simulink model "liquid_cooling_phase_a"  (R2026a)
settings: Solver=ode23t  StopTime=p.stopTime  MaxStep=1  RelTol=1e-5
model workspace (MAT data in the model file):
  p.Tambient_C = 25
  p.Tset_C = 40
  p.Tinitial_K = 298.15
  p.mChip = 0.16
  p.cpChip = 500
  p.mWater = 0.1
  p.cpWater = 4180
  p.RchipWater = 0.1
  p.Gpassive = 0.4
  p.Gfan = 5
  p.tauFan = 2
  p.Kp = 0.24
  p.Ki = 0.0012
  p.Kd = 0.5
  p.N = 1
  p.Qinitial = 20
  p.Qfinal = 40
  p.stepTime = 600
  p.stopTime = 1800
values from neighbouring files (symbols this model uses):
  p = getVariable(ws,'p'); p.Kp=g(1); p.Ki=g(2); p.Kd=g(3)    [apply_phase_a_pid_tuning.m]    (also in build_phase_a.m = phase_a_parameters(); phase_a_results.mat = ; pid_tuning_trials.mat = ; run_phase_a.m = getVariable(ws,'p'))
libraries: fl_lib x9, nesl_utility x5, slpidlib x1
settings Model: Creator=Aaron Xu  LastModifiedBy=Aaron Xu

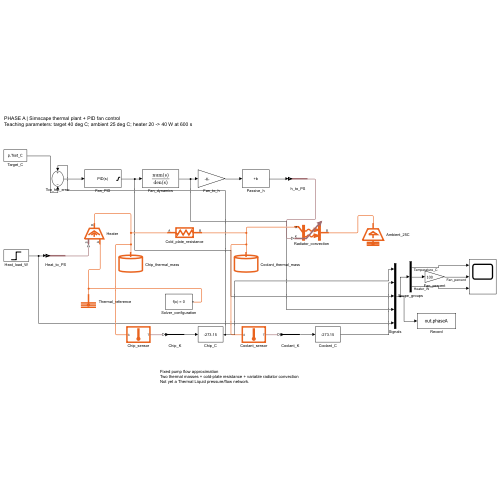
[thumbnail: Simulink's stored preview of the top-level diagram]
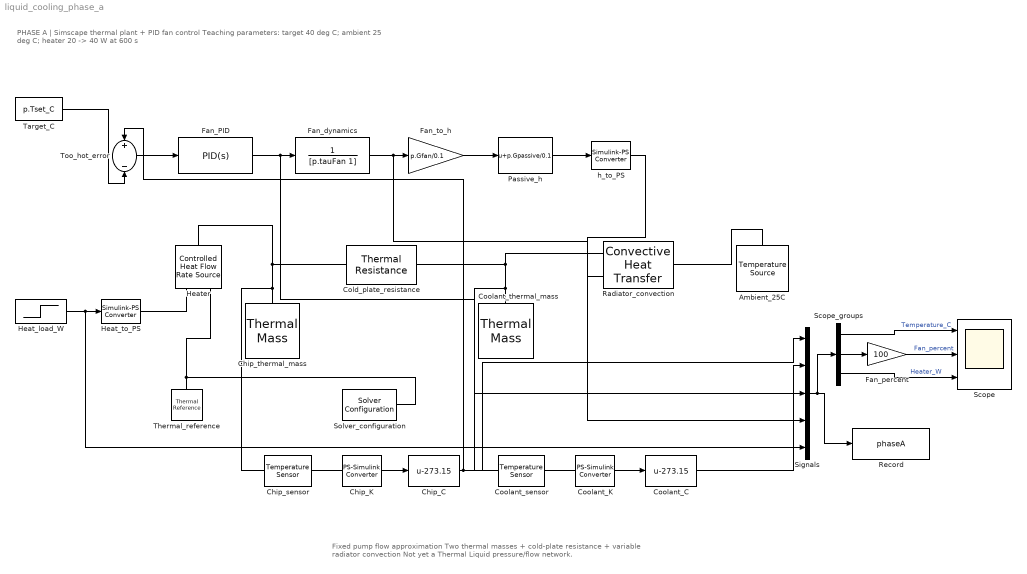
== system liquid_cooling_phase_a ==
  note: PHASE A | Simscape thermal plant + PID fan control
      | Teaching parameters: target 40 deg C; ambient 25 deg C; heater 20 -> 40 W at 600 s
  note: Fixed pump flow approximation
      | Two thermal masses + cold-plate resistance + variable radiator convection
      | Not yet a Thermal Liquid pressure/flow network.
  Ambient_25C : fl_lib/Thermal/Thermal Sources/Temperature Source  temperature=p.Tambient_C+273.15 K
  Chip_C : Bias  Bias=-273.15  SaturateOnIntegerOverflow=off
  Chip_K : nesl_utility/PS-Simulink Converter  PhysicalDomain=network_engine_domain  SubClassName=ps_output  LeftPortType=input  RightPortType=output  PseudoPeriodic=off  Frequencies=[]  VectorFormat=inherit  Unit=K  AffineConversion=off
  Chip_sensor : fl_lib/Thermal/Thermal Sensors/Temperature Sensor  temperature_measure=2
  Chip_thermal_mass : fl_lib/Thermal/Thermal Elements/Thermal Mass  mass_type=foundation.enum.constant_variable.constant  mass=p.mChip kg  sp_heat=p.cpChip J/(K*kg)  mass_min=1e-6 kg  num_ports=foundation.enum.numPorts2.one  m_specify=off  m_priority=High  m=1 kg  m_nominal_specify=off  m_nominal_value=1  m_nominal_unit=kg  T_specify=on  T_priority=High  T=p.Tinitial_K K  T_nominal_specify=off  T_nominal_value=1  T_nominal_unit=K  Q_specify=off  Q_priority=None  Q=0 W  Q_nominal_specify=off  Q_nominal_value=1  Q_nominal_unit=W
  Cold_plate_resistance : fl_lib/Thermal/Thermal Elements/Thermal Resistance  resistance=p.RchipWater K/W  T_specify=off  T_priority=None  T=0 K  T_nominal_specify=off  T_nominal_value=1  T_nominal_unit=K  Q_specify=off  Q_priority=None  Q=0 W  Q_nominal_specify=off  Q_nominal_value=1  Q_nominal_unit=W
  Coolant_C : Bias  Bias=-273.15  SaturateOnIntegerOverflow=off
  Coolant_K : nesl_utility/PS-Simulink Converter  PhysicalDomain=network_engine_domain  SubClassName=ps_output  LeftPortType=input  RightPortType=output  PseudoPeriodic=off  Frequencies=[]  VectorFormat=inherit  Unit=K  AffineConversion=off
  Coolant_sensor : fl_lib/Thermal/Thermal Sensors/Temperature Sensor  temperature_measure=2
  Coolant_thermal_mass : fl_lib/Thermal/Thermal Elements/Thermal Mass  mass_type=foundation.enum.constant_variable.constant  mass=p.mWater kg  sp_heat=p.cpWater J/(K*kg)  mass_min=1e-6 kg  num_ports=foundation.enum.numPorts2.one  m_specify=off  m_priority=High  m=1 kg  m_nominal_specify=off  m_nominal_value=1  m_nominal_unit=kg  T_specify=on  T_priority=High  T=p.Tinitial_K K  T_nominal_specify=off  T_nominal_value=1  T_nominal_unit=K  Q_specify=off  Q_priority=None  Q=0 W  Q_nominal_specify=off  Q_nominal_value=1  Q_nominal_unit=W
  Fan_PID : slpidlib/PID Controller  Controller=PID  Form=Parallel  TimeDomain=Continuous-time  UseExternalTs=off  SampleTime=-1  IntegratorMethod=Forward Euler  FilterMethod=Forward Euler  ControllerParametersSource=internal  P=p.Kp  I=p.Ki  UseKiTs=off  D=p.Kd  UseExternalDerivativeSource=off  N=p.N  UseFilter=on  TunerSelectOption=Transfer Function Based (PID Tuner App)  InitialConditionSource=internal  InitialConditionForIntegrator=0  InitialConditionForFilter=0  DifferentiatorICPrevScaledInput=0  ExternalReset=none  TrackingMode=off  Kt=1  LimitOutput=on  SatLimitsSource=internal  UpperSaturationLimit=1  LowerSaturationLimit=0  LinearizeAsGain=on  AntiWindupMode=clamping  Kb=1  LimitIntegrator=off  UpperIntegratorSaturationLimit=inf  LowerIntegratorSaturationLimit=-inf  POutMin=[]  POutMax=[]  IOutMin=[]  IOutMax=[]  DOutMin=[]  DOutMax=[]  NOutMin=[]  NOutMax=[]  SumOutMin=[]  SumOutMax=[]  SaturationOutMin=[]  SaturationOutMax=[]  PParamMin=[]  PParamMax=[]  IParamMin=[]  IParamMax=[]  DParamMin=[]  DParamMax=[]  NParamMin=[]  NParamMax=[]  KbParamMin=[]  KbParamMax=[]  KtParamMin=[]  KtParamMax=[]  KbOutMin=[]  KbOutMax=[]  KtOutMin=[]  KtOutMax=[]  IntegratorOutMin=[]  IntegratorOutMax=[]  FilterOutMin=[]  FilterOutMax=[]  SumI1OutMin=[]  SumI1OutMax=[]  SumI2OutMin=[]  SumI2OutMax=[]  SumI3OutMin=[]  SumI3OutMax=[]  SumI4OutMin=[]  SumI4OutMax=[]  SumDOutMin=[]  SumDOutMax=[]  DifferentiatorOutMin=[]  DifferentiatorOutMax=[]  FilterDiffOutCoefMin=[]  FilterDiffOutCoefMax=[]  ReciprocalOutMin=[]  ReciprocalOutMax=[]  SumDenOutMin=[]  SumDenOutMax=[]  SumNumOutMin=[]  SumNumOutMax=[]  DivideOutMin=[]  DivideOutMax=[]  UdiffTsProdOutMin=[]  UdiffTsProdOutMax=[]  NTsProdOutMin=[]  NTsProdOutMax=[]  UintegralTsProdOutMin=[]  UintegralTsProdOutMax=[]  UngainTsProdOutMin=[]  UngainTsProdOutMax=[]  ClampingZeroOutDataTypeStr=Inherit: Inherit via back propagation  ClampingZeroOutMin=[]  ClampingZeroOutMax=[]  FilterDenConstantOutDataTypeStr=Inherit: Inherit via back propagation  FilterDenConstantOutMin=[]  FilterDenConstantOutMax=[]  PCopyOutDataTypeStr=Inherit: Inherit via back propagation  PCopyOutMin=[]  PCopyOutMax=[]  NCopyOutDataTypeStr=Inherit: Inherit via back propagation  NCopyOutMin=[]  NCopyOutMax=[]  IntegratorContinuousStateAttributes=''  IntegratorStateMustResolveToSignalObject=off  IntegratorRTWStateStorageClass=Auto  FilterContinuousStateAttributes=''  FilterStateMustResolveToSignalObject=off  FilterRTWStateStorageClass=Auto  ParallelPVariant=InternalParameters  IdealPVariant=Disabled  IVariant=InternalParameters  DVariant=InternalParameters  IntegratorVariant=Continuous  SatVariant=Enabled  AWVariant=ContClampingParallel  PCopyVariant=Disabled  TRVariant=Disabled  FdbkBlocksVariant=Forward  IdealPFdbkVariant=Disabled  SatFdbkVariant=Disabled  DerivativeFilterVariant=ContFilter  NVariant=InternalParameters  NCopyVariant=Disabled  FilterICVariant=InternalICsFilter  IntegratorICVariant=InternalICs  ExternalResetVariant=Disabled  TRSumVariant=Passthrough  SumFdbkVariant=Disabled  SumVariant=Sum_PID  TsampFilterVariant=InternalTs  TsampNgainVariant=Passthrough  TsampIntegralVariant=Disabled_SignalSpec  ExternalSaturationOutDataTypeStr=Inherit: Same as second input  DerivativeSourceVariant=ErrorSignal  PreIntVariant=InternalPreInt
  Fan_dynamics : TransferFcn  Numerator=1  Denominator=[p.tauFan 1]
  Fan_percent : Gain  Gain=100
  Fan_to_h : Gain  Gain=p.Gfan/0.1
  Heat_load_W : Step  Time=p.stepTime  InitialValue=p.Qinitial  FinalValue=p.Qfinal  SampleTime=0
  Heat_to_PS : nesl_utility/Simulink-PS Converter  PhysicalDomain=network_engine_domain  SubClassName=ps_input  LeftPortType=input  RightPortType=output  PseudoPeriodic=off  Frequencies=[]  NoiseDistribution=none  NoiseParameters=[]  Unit=W  AffineConversion=off  FilteringAndDerivatives=provide  SimscapeFilterOrder=1  InputFilterTimeConstant=0.001  UdotUserProvided=0
  Heater : fl_lib/Thermal/Thermal Sources/Controlled Heat Flow Rate Source
  Passive_h : Bias  Bias=p.Gpassive/0.1  SaturateOnIntegerOverflow=off
  Radiator_convection : fl_lib/Thermal/Thermal Elements/Convective Heat Transfer  thermal_type=2  area=0.1 m^2  heat_tr_coeff=20 W/(K*m^2)  min_heat_tr_coeff=1e-3 W/(K*m^2)  T_specify=off  T_priority=None  T=0 K  T_nominal_specify=off  T_nominal_value=1  T_nominal_unit=K  Q_specify=off  Q_priority=None  Q=0 W  Q_nominal_specify=off  Q_nominal_value=1  Q_nominal_unit=W
  Record : ToWorkspace  VariableName=phaseA  SaveFormat=Timeseries  SampleTime=-1
  Scope : Scope  NumInputPorts=3
      settings: TimeSpan=1800  Title=Temperature: channel 1 = chip, channel 2 = coolant  ActiveDisplayYMinimum=24  ActiveDisplayYMaximum=46  YLabel=deg C
  Scope_groups : Demux  Outputs=[2 2 1]
  Signals : Mux  Inputs=5
  Solver_configuration : nesl_utility/Solver Configuration  PhysicalDomain=network_engine_domain  SubClassName=solver  LeftPortType=input  RightPortType=generic  Tones=[]  Harmonics=[]  SimulateNoise=off  Profile=off  UseLocalSampling=off  EnableSwitchedLinearOptims=on  FrequencyDomain=off  UseCCode=off  RelTol=0.001  AbsTol=0.001  MinStep=1e-09  ToWorkspace=off  RevertToSquareIcSolve=off  NumHomotopyIterations=100  PhasorMode=off  PhasorModeNumHarmonics=1  ConsistencySolver=NEWTON_XTOL_AFTER_FTOL  CanonicalOrdering=CANONICAL  OptimizeIntermediates=OPTIMIZED  IndexReductionMethod=DerivativeReplacement  DoDC=off  ResidualTolerance=1e-09  ConsistencyTolSource=GLOBAL  ConsistencyAbsTol=0.001  ConsistencyRelTol=0.001  ConsistencyTolFactor=0.001  UseLocalSolver=off  LocalSolverChoice=NE_BACKWARD_EULER_ADVANCER  ResolveIndetEquations=on  FunctionEvalNumThread=1  LocalSolverSampleTime=0.001  DoFixedCost=off  MaxNonlinIter=3  MaxModeIter=2  ComputeImpulses=off  ImpulseIterations=2  LinearAlgebra=auto  LinearAlgebraNumThread=0  EquationFormulation=NE_TIME_EF  DelaysMemoryBudget=1024  AutomaticFiltering=on  FilteringTimeConstant=0.001  PartitionStorageMethod=AS_NEEDED  PartitionMemoryBudget=1024  PartitionMethod=ROBUST  MultibodyUseLocalSolver=off  MultibodyLocalSolverChoice=ODE1  MultibodyLocalSolverSampleTime=0.001
  Target_C : Constant  Value=p.Tset_C
  Thermal_reference : fl_lib/Thermal/Thermal Elements/Thermal Reference
  Too_hot_error : Sum  Inputs=+-
  h_to_PS : nesl_utility/Simulink-PS Converter  PhysicalDomain=network_engine_domain  SubClassName=ps_input  LeftPortType=input  RightPortType=output  PseudoPeriodic=off  Frequencies=[]  NoiseDistribution=none  NoiseParameters=[]  Unit=W/(m^2*K)  AffineConversion=off  FilteringAndDerivatives=provide  SimscapeFilterOrder=1  InputFilterTimeConstant=0.001  UdotUserProvided=0
  wires:
  Target_C/1 -> Too_hot_error/2
  Chip_C/1 -> Too_hot_error/1, Signals/1
  Too_hot_error/1 -> Fan_PID/1
  Fan_PID/1 -> Fan_dynamics/1, Signals/3
  Fan_dynamics/1 -> Fan_to_h/1, Signals/4
  Fan_to_h/1 -> Passive_h/1
  Passive_h/1 -> h_to_PS/1
  Heat_load_W/1 -> Heat_to_PS/1, Signals/5
  Chip_K/1 -> Chip_C/1
  Coolant_K/1 -> Coolant_C/1
  Coolant_C/1 -> Signals/2
  Signals/1 -> Record/1, Scope_groups/1
  Scope_groups/1 -> Scope/1  "Temperature_C"
  Scope_groups/2 -> Fan_percent/1
  Fan_percent/1 -> Scope/2  "Fan_percent"
  Scope_groups/3 -> Scope/3  "Heater_W"
  connections:
  Heat_to_PS/RConn1 -- Heater/RConn1
  Thermal_reference/LConn1 -- Heater/RConn2 -- Solver_configuration/RConn1
  Heater/LConn1 -- Chip_thermal_mass/LConn1 -- Chip_sensor/LConn1 -- Cold_plate_resistance/LConn1
  Cold_plate_resistance/RConn1 -- Coolant_thermal_mass/LConn1 -- Coolant_sensor/LConn1 -- Radiator_convection/LConn1
  h_to_PS/RConn1 -- Radiator_convection/LConn2
  Radiator_convection/RConn1 -- Ambient_25C/LConn1
  Chip_sensor/RConn1 -- Chip_K/LConn1
  Coolant_sensor/RConn1 -- Coolant_K/LConn1
